simulink model "tractor_mu"  (R2022b)
settings: Solver=FixedStepDiscrete  StartTime=0.0  StopTime=20  FixedStep=0.001  RelTol=1e-3
model workspace (MAT data in the model file):
  P : object (value not decoded)
  w_2 : Simulink.Parameter (value not decoded)
undefined symbols (not defined in the file): A, a, B, b, C, D, DiscIntNeverNeededParam, Iz, K, k1, K1, k2, K2, L1, L2, m, magnitude, Phi, Sample_time, Steer_Ratio
libraries: simulink x26, slpidlib x13, Solver_SF x1, dsparch4 x1
(part 6 of 7)

== matlab function tractor_mu/加速度滑模观测/MATLAB Function1 ==
  data: a_xm input; a_xc output; a_ym input; v_xGPS input; v_yGPS input; gamma_c input; GPS_update_flag input; a_yc output; e_ax_est output; e_ay_est output; reset input
function [a_xc, a_yc, e_ax_est, e_ay_est] = accel_SMO_correction(a_xm, a_ym, v_xGPS, v_yGPS, gamma_c, GPS_update_flag, reset)
% 加速度滑模观测器校正
% 输入：
%   a_xm, a_ym      - INS测量的加速度 (m/s^2)
%   v_xGPS, v_yGPS  - GPS测量的速度 (m/s)
%   gamma_c         - 校正后的横摆角速度 (rad/s)
%   GPS_update_flag - GPS更新标志 (1=有新数据)
%   reset           - 复位信号
% 输出：
%   a_xc, a_yc      - 校正后的加速度
%   e_ax_est, e_ay_est - 估计的加速度偏差

% 采样时间
dt = 0.001;     % 仿真步长
DT = 0.05;      % GPS采样周期

% 滑模观测器增益（需根据实际调参）
persistent k1 k2 lambda1 lambda2
if isempty(k1)
    k1 = 5;       % 速度误差增益
    k2 = 5;
    lambda1 = 0.5; % 加速度偏差增益
    lambda2 = 0.5;
end

% 持久变量（状态记忆）
persistent v_xI v_yI e_ax e_ay initialized
persistent a_xm_sum a_ym_sum sum_count

if isempty(initialized) || reset
    v_xI = 0;      % INS积分速度 x
    v_yI = 0;      % INS积分速度 y
    e_ax = 0;      % 加速度偏差估计 x
    e_ay = 0;      % 加速度偏差估计 y
    a_xm_sum = 0;  % 加速度累加（用于GPS周期内求和）
    a_ym_sum = 0;
    sum_count = 0;
    initialized = true;
end

% 累加加速度（对应论文中的求和项）
a_xm_sum = a_xm_sum + a_xm;
a_ym_sum = a_ym_sum + a_ym;
sum_count = sum_count + 1;

% 速度积分（考虑横摆角速度耦合，对应式3-10）
% v_xI(k+1) = v_xI(k) + dt*a_xm + DT*(v_yI*gamma_c - e_ax - n_ax)
% 简化：每步用校正后的加速度积分
a_xc_temp = a_xm - e_ax;
a_yc_temp = a_ym - e_ay;

% 考虑横摆角速度耦合的速度更新
v_xI = v_xI + dt * (a_xc_temp + v_yI * gamma_c);
v_yI = v_yI + dt * (a_yc_temp - v_xI * gamma_c);

% GPS更新时刻：执行滑模校正
if GPS_update_flag == 1
    % 速度误差（观测残差）
    e_vx = v_xI - v_xGPS;
    e_vy = v_yI - v_yGPS;
    
    % 滑模切换函数
    s_x = sign(e_vx);
    s_y = sign(e_vy);
    
    % 也可用饱和函数避免抖振
    % epsilon = 0.1;
    % s_x = sat_func(e_vx, epsilon);
    % s_y = sat_func(e_vy, epsilon);
    
    % 速度校正（直接用GPS速度重置，或软校正）
    % 软校正方式：
    v_xI = v_xI - k1 * DT * s_x;
    v_yI = v_yI - k2 * DT * s_y;
    
    % 加速度偏差更新（滑模观测器核心）
    e_ax = e_ax + lambda1 * DT * s_x;
    e_ay = e_ay + lambda2 * DT * s_y;
    
    % 限幅防止发散
    e_ax = max(min(e_ax, 2), -2);
    e_ay = max(min(e_ay, 2), -2);
    
    % 清零累加器
    a_xm_sum = 0;
    a_ym_sum = 0;
    sum_count = 0;
end

% 输出校正后的加速度（式3-12）
a_xc = a_xm - e_ax;
a_yc = a_ym - e_ay;

% 输出偏差估计（用于调试）
e_ax_est = e_ax;
e_ay_est = e_ay;

end

% 饱和函数（可选，减少抖振）
function y = sat_func(x, epsilon)
    if abs(x) <= epsilon
        y = x / epsilon;
    else
        y = sign(x);
    end
end

== matlab function tractor_mu/质心侧偏角观测/MATLAB Function ==
  data: x_hat input; x_dot output; u input; z_meas input; z_hat output
function [x_dot, z_hat] = fcn(x_hat, u, z_meas)

    % === 车辆物理参数 ===
    mv = 18530;       % Vehicle total mass (kg)
    Izz = 67536;      % Second moment of mass (kg m^2)
    L1 = 2.043;        % CG to front axle (m)
    L2 = 1.362;        % CG to rear axle (m)
    Cf1 = 304828 * 2;     % Front cornering stiffness (N/rad) - 对应图中 C_F\delta^1
    Cf2 = 417040 * 2;     % Rear cornering stiffness (N/rad) - 对应图中 C_F\delta^2

    % === 观测器参数===
    Lambda = [100, 0;    % 增益矩阵 (3x2)
          0, 100;    
          0, 1000];   
    lambda_param = 1;
    Ts = 0.001;           % 离散采样时间 (Discrete Sample Time)

    % === 1. 解包状态变量和输入 ===
    % x_hat = [Vg_est; delta_est; r_est] 
    x1 = x_hat(1); % V_G
    x2 = x_hat(2); % delta (侧偏角)
    x3 = x_hat(3); % psi_dot (横摆角速度)

    % u = [beta; Fl1; Fl2]
    u1 = u(1); % beta
    u2 = u(2); % Fl1
    u3 = u(3); % Fl2
    
    % 防止分母为0
    if abs(x1) < 0.1
        x1 = 0.1; 
    end

    % === 2. 计算估计的输出 z_hat  ===
    % z = [Vg; psi_dot]
    h_NL = [x1; x3]; 
    z_hat = h_NL;

    % === 3. 计算观测误差 (z - z_hat) ===
    error = z_meas - z_hat;

    % === 4. 计算 Sign_eq 函数 ===
    sign_term = (2/pi) * atan(lambda_param * error);

    % === 5. 计算非线性函数 ===
    term1_1 = (1/mv) * (u2 * cos(x2 - u1) + u3 * cos(x2));
    term1_2 = (1/mv) * Cf2 * (-x2 + L2*x3/x1) * sin(x2);
    term1_3 = (1/mv) * Cf1 * (u1 - x2 - L1*x3/x1) * sin(x2 - u1);
    
    dx1_val = term1_1 + term1_2 + term1_3;

    term2_1 = 1/(mv*x1) * (u2 * sin(u1 - x2) - u3 * sin(x2)) ;
    term2_2 = 1/(mv*x1) * Cf1 * (u1 - x2 - L1*x3/x1) * cos(u1 - x2);
    term2_3 = 1/(mv*x1) * Cf2 * (-x2 + L2*x3/x1) * cos(x2) - x3;
    
    dx2_val = term2_1 + term2_2 + term2_3;

    term3_1 = (1/Izz) * ( L1 * u2 * sin(u1) - L2 * Cf2 * (-x2 + L2*x3/x1) ); 
    term3_2 = (1/Izz) * L1 * Cf1 * (u1 - x2 - L1*x3/x1) * cos(u1);
    
    dx3_val = term3_1 + term3_2;
    
    f_NL = [dx1_val; dx2_val; dx3_val];

    % === 6. 最终观测器状态导数 ===
    % x_hat_dot = f_NL(x_hat, u) + Lambda * sign_eq(z - z_hat)
    x_dot = f_NL + Lambda * sign_term;
end

== matlab function tractor_mu/软土扭矩分配/牵引功率目标计算 ==
  data: dt_s input; drawbar_power_w output; wheel_omegas_radps input; previous_applied_torques_n_m input; longitudinal_speed_mps input; implement_force_x_n input; wheel_power_w output; phi_raw output; filtered_phi output; filtered_normalized_phi output; lambda_est output; objective_valid output
function [drawbar_power_w, wheel_power_w, phi_raw, filtered_phi, filtered_normalized_phi, lambda_est, objective_valid] = MF_TractionEfficiencyObjective(dt_s, wheel_omegas_radps, previous_applied_torques_n_m, longitudinal_speed_mps, implement_force_x_n)

% 牵引效率目标函数计算模块
%
% 本模块计算牵引效率相关的在线优化目标：
% eta = P_drawbar / P_wheel
%
% 并构造 Dinkelbach 差值型目标：
% phi = P_drawbar - lambda * P_wheel

persistent has_filtered_power filtered_drawbar_power_state filtered_wheel_power_state
persistent has_filtered_phi filtered_phi_state filtered_normalized_phi_state
persistent lambda_state

if isempty(has_filtered_power)

    has_filtered_power = 0.0;
    filtered_drawbar_power_state = 0.0;
    filtered_wheel_power_state = 0.0;

    has_filtered_phi = 0.0;
    filtered_phi_state = 0.0;
    filtered_normalized_phi_state = 0.0;

    lambda_state = 0.0;
end

%% 输入整理

dt = max(double(dt_s), 0.0);
omegas = row4_local(wheel_omegas_radps);
applied_torques = row4_local(previous_applied_torques_n_m);

vx = double(longitudinal_speed_mps);
implement_force = double(implement_force_x_n);

%% 轮端输入功率计算

% 轮端输入功率 P_wheel = sum(T_i * omega_i)。
% 只保留非负驱动功率，避免制动功率或异常信号影响牵引效率评价。
wheel_drive_powers = zeros(1, 4);

for index = 1:4
    wheel_drive_powers(index) = max(0.0, applied_torques(index) * abs(omegas(index)));
end

wheel_power_w = sum(wheel_drive_powers);

%% 有效牵引功率计算

% 农具阻力方向通常与车辆行驶方向相反。
% 前进时，如果 implement_force 为负，则 -implement_force 为有效牵引阻力。
% 倒车时符号相反。
if vx > 0.08
    drawbar_force = max(0.0, -implement_force);
elseif vx < -0.08
    drawbar_force = max(0.0, implement_force);
else
    drawbar_force = 0.0;
end

drawbar_power_w = drawbar_force * abs(vx);

%% 目标函数有效性判断

% 轮端输入功率过低或车速过低时，牵引效率计算不可靠。
objective_valid = wheel_power_w >= 100.0 && abs(vx) > 0.08;

%% 功率滤波

alpha_objective = first_order_alpha_local(dt, 0.7);

if has_filtered_power <= 0.5 || ~objective_valid

    filtered_drawbar_power_state = drawbar_power_w;
    filtered_wheel_power_state = wheel_power_w;
    has_filtered_power = 1.0;

else

    filtered_drawbar_power_state = filtered_drawbar_power_state + ...
        alpha_objective * (drawbar_power_w - filtered_drawbar_power_state);

    filtered_wheel_power_state = filtered_wheel_power_state + ...
        alpha_objective * (wheel_power_w - filtered_wheel_power_state);

    has_filtered_power = 1.0;
end

%% lambda 牵引效率参数更新

if objective_valid

    eta_instant = drawbar_power_w / max(wheel_power_w, 1.0e-9);

    alpha_lambda = first_order_alpha_local(dt, 1.0);

    lambda_state = lambda_state + alpha_lambda * (eta_instant - lambda_state);
end

lambda_est = lambda_state;

%% Dinkelbach 差值型性能指标

phi_raw = drawbar_power_w - lambda_est * wheel_power_w;

% 归一化性能指标，用于降低功率量级变化对极值寻优的影响。
normalized_phi = phi_raw / max(abs(wheel_power_w), 1000.0);

%% 性能指标滤波

if has_filtered_phi <= 0.5 || ~objective_valid

    filtered_phi_state = phi_raw;
    filtered_normalized_phi_state = normalized_phi;
    has_filtered_phi = 1.0;

else

    filtered_phi_state = filtered_phi_state + ...
        alpha_objective * (phi_raw - filtered_phi_state);

    filtered_normalized_phi_state = filtered_normalized_phi_state + ...
        alpha_objective * (normalized_phi - filtered_normalized_phi_state);

    has_filtered_phi = 1.0;
end

filtered_phi = filtered_phi_state;
filtered_normalized_phi = filtered_normalized_phi_state;

end


function output = row4_local(values)

% 将输入信号整理为 1×4 行向量。

input_values = double(values);
output = zeros(1, 4);

for index = 1:4
    output(index) = input_values(index);
end

end


function alpha = first_order_alpha_local(dt, time_constant_s)

% 一阶低通滤波系数：
% y(k) = y(k-1) + alpha * [u(k) - y(k-1)]

if dt <= 0.0 || time_constant_s <= 0.0
    alpha = 1.0;
else
    alpha = dt / (time_constant_s + dt);
end

end

== matlab function tractor_mu/软土扭矩分配/四轮目标滑移率计算 ==
  data: current_time_s input; adaptive_targets output; dt_s input; filtered_normalized_phi input; objective_valid input; kappa_valid input; target_base_out output; gradient_estimates output
function [adaptive_targets, target_base_out, gradient_estimates] = MF_AdaptiveSlipTarget4W(current_time_s, dt_s, filtered_normalized_phi, objective_valid, kappa_valid)

% 四轮自适应目标滑移率生成模块
%
% 采用多变量极值寻优思想，对四个车轮的目标滑移率进行独立更新。
%
% 四轮顺序：
% 1：左前轮
% 2：右前轮
% 3：左后轮
% 4：右后轮

persistent target_base_state gradient_state

if isempty(target_base_state)

    % 初始目标滑移率仍保持原前后轴标定值。
    target_base_state = [0.078, 0.078, 0.128, 0.128];

    % 四轮梯度估计初值。
    gradient_state = zeros(1, 4);
end

%% 输入整理

time_s = double(current_time_s);
dt = max(double(dt_s), 0.0);
normalized_phi = double(filtered_normalized_phi);
valid_vec = row4_local(kappa_valid);

%% 极值寻优参数

% 四轮扰动频率，单位 Hz。
frequencies = [0.7, 0.9, 1.1, 1.3];

% 目标滑移率扰动幅值。
perturb_amp = 0.002;

% 目标滑移率基值自适应增益。
adapt_gain = 0.0006;

% 目标滑移率允许范围。
target_min = 0.03;
target_max = 0.25;

% 梯度低通滤波系数。
alpha_gradient = first_order_alpha_local(dt, 0.8);

%% 是否允许更新目标基值

update_enabled = double(objective_valid) > 0.5 && all(valid_vec > 0.5);

%% 生成四轮扰动信号

sine_signals = zeros(1, 4);

for index = 1:4
    sine_signals(index) = sin(2.0 * pi * frequencies(index) * time_s);
end

%% 梯度估计与目标基值更新

if update_enabled

    for index = 1:4

        % 极值寻优解调。
        % 性能指标与扰动信号相乘，用于估计该轮目标滑移率变化对牵引效率目标的边际影响。
        gradient_raw = 2.0 * normalized_phi * sine_signals(index) / perturb_amp;

        % 梯度估计低通滤波。
        gradient_state(index) = gradient_state(index) + ...
            alpha_gradient * (gradient_raw - gradient_state(index));

        % 限制每个采样周期目标滑移率基值的最大变化量。
        max_delta = 0.003 * dt;

        target_delta = clamp_local(adapt_gain * gradient_state(index) * dt, -max_delta, max_delta);

        % 更新目标滑移率基值。
        target_base_state(index) = clamp_local(target_base_state(index) + target_delta, target_min, target_max);
    end
end

%% 输出四轮目标滑移率

adaptive_targets = zeros(1, 4);

for index = 1:4

    % 最终目标 = 基值 + 小幅正弦扰动。
    adaptive_targets(index) = clamp_local( ...
        target_base_state(index) + perturb_amp * sine_signals(index), ...
        target_min, target_max);
end

% 调试输出，可在 Simulink 中不连接。
target_base_out = target_base_state;
gradient_estimates = gradient_state;

end


function output = row4_local(values)

% 将输入信号整理为 1×4 行向量。

input_values = double(values);
output = zeros(1, 4);

for index = 1:4
    output(index) = input_values(index);
end

end


function alpha = first_order_alpha_local(dt, time_constant_s)

% 一阶低通滤波系数。

if dt <= 0.0 || time_constant_s <= 0.0
    alpha = 1.0;
else
    alpha = dt / (time_constant_s + dt);
end

end


function value = clamp_local(value_in, lower, upper)

% 数值限幅函数。

value = min(max(double(value_in), double(lower)), double(upper));

end

== matlab function tractor_mu/牵引效率计算/计算平均边际贡献 ==
  data: v_all input; phi output
function phi = shapley_calc(v_all)

% 输入:
% v_all: 16x1
%
% 子集顺序:
%
% 1  -> []
% 2  -> [1]
% 3  -> [2]
% 4  -> [3]
% 5  -> [4]
% 6  -> [1 2]
% 7  -> [1 3]
% 8  -> [1 4]
% 9  -> [2 3]
% 10 -> [2 4]
% 11 -> [3 4]
% 12 -> [1 2 3]
% 13 -> [1 2 4]
% 14 -> [1 3 4]
% 15 -> [2 3 4]
% 16 -> [1 2 3 4]
%
% 输出:
% phi = [FL; FR; RL; RR]

%% 平移法消除负值

v_min = min(v_all);

if v_min < 0
    v_all = v_all - v_min;
end

%% 参数

n = 4;

fact = factorial(0:n);

phi = zeros(4,1);

%% 联盟定义

coalitions = [...
    0 0 0 0;  % 1
    1 0 0 0;  % 2
    0 1 0 0;  % 3
    0 0 1 0;  % 4
    0 0 0 1;  % 5
    1 1 0 0;  % 6
    1 0 1 0;  % 7
    1 0 0 1;  % 8
    0 1 1 0;  % 9
    0 1 0 1;  % 10
    0 0 1 1;  % 11
    1 1 1 0;  % 12
    1 1 0 1;  % 13
    1 0 1 1;  % 14
    0 1 1 1;  % 15
    1 1 1 1]; % 16

%% Shapley计算

for i = 1:n

    for idx = 1:16

        S = coalitions(idx,:);

        % 若联盟中已有玩家i
        if S(i) == 1
            continue;
        end

        % 联盟大小
        k = sum(S);

        % 权重
        w = fact(k+1) * fact(n-k) / fact(n+1);

        % v(S)
        v_S = v_all(idx);

        % 构造 S∪{i}
        S_with_i = S;
        S_with_i(i) = 1;

        %% 查找 S∪{i} 对应索引

        idx_Si = 1;

        for j = 1:16

            if isequal(coalitions(j,:), S_with_i)

                idx_Si = j;
                break;

            end

        end

        % v(S∪{i})
        v_Si = v_all(idx_Si);

        % Shapley累加
        phi(i) = phi(i) + w * (v_Si - v_S);

    end

end

phi_min = min(phi);

if phi_min < 0
    phi = phi - phi_min;
end

end

== matlab function tractor_mu/协同博弈扭矩分配/MATLAB Function ==
  data: v input; alpha output
function alpha = fcn(v)

if v < 0.5
    alpha = 0;
elseif v < 5
    alpha = (v - 0.5)/(5 - 0.5);
else
    alpha = 1;
end

== matlab function tractor_mu/牵引效率计算/MATLAB Function3 ==
  data: Fx input; V_all output; Vx input; T input; uF input; mu input; Fz input; slip input; Mz_ref input; Traction_all output; lamdaN_all output; lamda_all output; Mz_all output
function [V_all,Traction_all,lamdaN_all,lamda_all,Mz_all] = shapley_value_all(...
Fx,...
Vx,...
T,...
uF,...
mu,...
Fz,...
slip,...
Mz_ref)

%% 参数

kf = 3;   % 前轮牵引权重
kr = 6;   % 后轮牵引权重

w1 = 100000;  % 滑转率损失权重
w2 = 5000;    % 附着利用率均衡权重
w3 = 0.0001;  % 横摆稳定损失权重

% 半轮距
bf = 2.39/2;
br = 2.33/2;

%% 初始化

V_all = zeros(16,1);
Traction_all = zeros(16,1);
lamdaN_all = zeros(16,1);
lamda_all = zeros(16,1);
Mz_all = zeros(16,1);

%% 16个联盟

coalitions = [...
    0 0 0 0;  % 空集-1
    1 0 0 0;  % 2
    0 1 0 0;  % 3
    0 0 1 0;  % 4
    0 0 0 1;  % 5
    1 1 0 0;  % 6
    1 0 1 0;  % 7
    1 0 0 1;  % 8
    0 1 1 0;  % 9
    0 1 0 1;  % 10
    0 0 1 1;  % 11
    1 1 1 0;  % 12
    1 1 0 1;  % 13
    1 0 1 1;  % 14
    0 1 1 1;  % 15
    1 1 1 1];  % 16

%% 遍历所有联盟

for k = 1:16

    coalition = coalitions(k,:)';

    %% 联盟数据

    Fx_s    = Fx    .* coalition;
    T_s     = T     .* coalition;
    uF_s    = uF   .* coalition;
    mu_s    = mu    .* coalition;
    Fz_s    = Fz    .* coalition;
    slip_s  = slip   .* coalition;

    %% 1 牵引能力项

    F_front = uF_s(1) + uF_s(2);
    F_rear  = uF_s(3) + uF_s(4);

    traction_term = ...
        kf * F_front + ...
        kr * F_rear;

    %% 2 滑转率损失

    
    % 只保留联盟中的驱动轮滑转率
    slip_active = abs(slip_s);

    % 防止空集导致 max([]) 问题
if sum(coalition) == 0

    lamdaN = 0;

else

    % 最大滑转率
    slip_max = max(slip_active);

    % 四次方强化惩罚
    lamdaN = slip_max^4;

end


    %% 3 附着利用率

    lambda_term = 0;

    for i = 1:4

        if coalition(i) == 1

            denom = uF_s(i);

            if abs(denom) > 1e-6

                lambda_i = Fx_s(i) / denom;

                % 平方强化
                lambda_term = ...
                    lambda_term + lambda_i^2;

            end

        end

    end

    %% 4 横摆力矩

    Mz = ...
        (-Fx_s(1) + Fx_s(2)) * bf + ...
        (-Fx_s(3) + Fx_s(4)) * br;

    %Mz = 

    %% 5 价值函数

    V_all(k) = ...
        traction_term ...
        - w1 * lamdaN ...
        + w2 * lambda_term ...
        - w3 * (Mz - Mz_ref)^2;

    Traction_all(k) = traction_term;
    lamdaN_all(k) = -w1 * lamdaN;
    lamda_all(k) = w2 * lambda_term;
    Mz_all(k) = - w3 * (Mz - Mz_ref)^2;

end

end

== matlab function tractor_mu/软土分配策略/MATLAB Function ==
  data: wheel_speeds_rpm input; selected_torques_n_m output; front_steer_angles_deg input; longitudinal_speed_mps input; applied_torques_n_m input; drive_torque_enabled input; baseline_torques_n_m input; wheel_torque_limits_n_m input; control_kappa output; filtered_kappa output; kappa_valid output; adaptive_targets output; cbf_torque_upper_bounds output; cbf_active output; nominal_torques_n_m output; soft_diag output
function [selected_torques_n_m, control_kappa, filtered_kappa, kappa_valid, adaptive_targets, cbf_torque_upper_bounds, cbf_active, nominal_torques_n_m, soft_diag] = shiche_soft_soil_adaptive_allocation(wheel_speeds_rpm, front_steer_angles_deg, longitudinal_speed_mps, applied_torques_n_m, drive_torque_enabled, baseline_torques_n_m, wheel_torque_limits_n_m)
%SHICHE_SOFT_SOIL_ADAPTIVE_ALLOCATION Real-vehicle soft-soil clamp allocator.
%
% MATLAB Function block version for VCU code generation. All numeric states,
% constants, intermediate arrays, and outputs are single precision.
%
% Wheel vector order is fixed as a 4x1 column:
%   [L1, R1, L2, R2] = [left-front, right-front, left-rear, right-rear]
%
% This block assumes an upstream load-based/basic four-wheel torque allocator
% already exists. baseline_torques_n_m is used as the reproducible anchor
% allocation. This real-vehicle version intentionally avoids QP, matrix solves,
% and active-set enumeration: it applies slip-tracking torque correction and
% then clamps each wheel by the CBF safety upper bound.
%
% Inputs:
%   wheel_speeds_rpm        single, 4x1 wheel speeds in rpm, [L1 R1 L2 R2].
%   front_steer_angles_deg  single, [Steer_L1 Steer_R1] in deg, or one scalar.
%   longitudinal_speed_mps  single, vehicle longitudinal speed in m/s.
%   applied_torques_n_m     single, 4x1 actual or one-step delayed applied wheel
%                           torques in N*m, [L1 R1 L2 R2].
%   drive_torque_enabled    single flag, >0.5 enables adaptive update and CBF.
%   baseline_torques_n_m    single, 4x1 upstream basic allocation in N*m.
%   wheel_torque_limits_n_m single, 4x1 nonnegative wheel torque limits in N*m.
%
% Outputs are single. kappa_valid and cbf_active are 0/1 single flags. soft_diag
% has 26 entries:
%   1:6   front target, rear target, simplified allocator status, total torque
%         reduction by CBF clamp, baseline total torque, selected total torque
%   7:10  filtered slip derivatives
%   11:14 slip input gains
%   15:18 slip disturbance estimates
%   19:22 disturbance margins
%   23:26 wheel surface speeds

persistent has_filtered filtered_state filtered_dot_state disturbance_state

if isempty(has_filtered)
    has_filtered = zeros(4, 1, 'single');
    filtered_state = zeros(4, 1, 'single');
    filtered_dot_state = zeros(4, 1, 'single');
    disturbance_state = zeros(4, 1, 'single');
end

dt = single(0.02);
wheel_speeds = column4_local(wheel_speeds_rpm);
front_steers = front_steer_pair_local(front_steer_angles_deg);
control_vx = single(longitudinal_speed_mps);
applied_torques = column4_local(applied_torques_n_m);
base_torques = column4_local(baseline_torques_n_m);
wheel_limits = column4_local(wheel_torque_limits_n_m);
drive_enabled = single(drive_torque_enabled) > single(0.5);

for index = 1:4
    wheel_limits(index) = max(single(0.0), wheel_limits(index));
    base_torques(index) = clamp_local(base_torques(index), single(0.0), wheel_limits(index));
end

[control_kappa, filtered_kappa, kappa_valid, dot_kappa, rolling_speeds, wheel_omegas, surface_speeds, has_filtered, filtered_state, filtered_dot_state] = ...
    update_slip_local(wheel_speeds, front_steers, control_vx, dt, has_filtered, filtered_state, filtered_dot_state);

front_target_base = single(0.078);
rear_target_base = single(0.128);
adaptive_targets = zeros(4, 1, 'single');
adaptive_targets(1) = front_target_base;
adaptive_targets(2) = front_target_base;
adaptive_targets(3) = rear_target_base;
adaptive_targets(4) = rear_target_base;

input_gains = input_gains_local(kappa_valid, rolling_speeds, wheel_omegas);
[disturbance_state, disturbance_margins] = update_disturbance_local(kappa_valid, dot_kappa, input_gains, applied_torques, dt, disturbance_state);

front_error = axle_slip_error_local(filtered_kappa, kappa_valid, adaptive_targets(1), 1);
rear_error = axle_slip_error_local(filtered_kappa, kappa_valid, adaptive_targets(3), 2);

nominal_torques_n_m = zeros(4, 1, 'single');
cbf_torque_upper_bounds = zeros(4, 1, 'single');
cbf_active = zeros(4, 1, 'single');
for index = 1:4
    gain = input_gains(index);
    if drive_enabled && kappa_valid(index) > single(0.5) && isfinite(gain)
        if index <= 2
            axle_error = front_error;
        else
            axle_error = rear_error;
        end
        torque_delta = clamp_local(-single(20500.0) * axle_error, -single(2600.0), single(2600.0));
        nominal = base_torques(index) + torque_delta;
    else
        nominal = base_torques(index);
    end
    nominal_torques_n_m(index) = clamp_local(nominal, single(0.0), wheel_limits(index));

    if drive_enabled && kappa_valid(index) > single(0.5) && isfinite(gain)
        upper = (single(15.0) * (single(0.25) - filtered_kappa(index)) - disturbance_state(index) - disturbance_margins(index)) / gain;
        if ~isfinite(upper)
            upper = wheel_limits(index);
        end
        upper = clamp_local(upper, single(0.0), wheel_limits(index));
    else
        upper = wheel_limits(index);
    end
    cbf_torque_upper_bounds(index) = upper;
    if upper < base_torques(index) - single(1.0e-6)
        cbf_active(index) = single(1.0);
    end
end

selected_torques_n_m = zeros(4, 1, 'single');
for index = 1:4
    selected_torques_n_m(index) = clamp_local(nominal_torques_n_m(index), single(0.0), cbf_torque_upper_bounds(index));
end

allocator_status = single(1.0);
total_torque_reduction = sum(nominal_torques_n_m - selected_torques_n_m);
baseline_total_torque = sum(base_torques);
selected_total_torque = sum(selected_torques_n_m);

soft_diag = zeros(26, 1, 'single');
soft_diag(1) = front_target_base;
soft_diag(2) = rear_target_base;
soft_diag(3) = allocator_status;
soft_diag(4) = total_torque_reduction;
soft_diag(5) = baseline_total_torque;
soft_diag(6) = selected_total_torque;
for index = 1:4
    soft_diag(6 + index) = dot_kappa(index);
    soft_diag(10 + index) = input_gains(index);
    soft_diag(14 + index) = disturbance_state(index);
    soft_diag(18 + index) = disturbance_margins(index);
    soft_diag(22 + index) = surface_speeds(index);
end
end

function [raw_kappa, filtered_kappa, valid, dot_kappa, rolling_speeds, omegas, surface_speeds, has_filtered_out, filtered_state_out, filtered_dot_out] = update_slip_local(wheel_speeds, front_steers, vx_mps, dt, has_filtered_in, filtered_state_in, filtered_dot_in)
rpm_to_rad = single(2.0) * single(pi) / single(60.0);
radii = zeros(4, 1, 'single');
radii(1) = single(0.834);
radii(2) = single(0.834);
radii(3) = single(0.94);
radii(4) = single(0.94);
speed_abs = abs(single(vx_mps));
steer_l = front_steers(1) * single(pi) / single(180.0);
steer_r = front_steers(2) * single(pi) / single(180.0);
rolling_speeds = zeros(4, 1, 'single');
rolling_speeds(1) = abs(speed_abs * cos(steer_l));
rolling_speeds(2) = abs(speed_abs * cos(steer_r));
rolling_speeds(3) = speed_abs;
rolling_speeds(4) = speed_abs;
omegas = abs(single(wheel_speeds)) * rpm_to_rad;
surface_speeds = radii .* omegas;

raw_kappa = zeros(4, 1, 'single');
filtered_kappa = zeros(4, 1, 'single');
dot_kappa = zeros(4, 1, 'single');
valid = zeros(4, 1, 'single');
has_filtered_out = has_filtered_in;
filtered_state_out = filtered_state_in;
filtered_dot_out = filtered_dot_in;
for index = 1:4
    raw_kappa(index) = single(NaN);
    filtered_kappa(index) = single(NaN);
end

alpha_kappa = first_order_alpha_local(dt, single(0.04));
alpha_dot = first_order_alpha_local(dt, single(0.08));
for index = 1:4
    is_valid = speed_abs >= single(0.08) && surface_speeds(index) >= single(0.20) && isfinite(rolling_speeds(index)) && isfinite(surface_speeds(index));
    if is_valid
        valid(index) = single(1.0);
        raw_value = single(1.0) - rolling_speeds(index) / surface_speeds(index);
        raw_kappa(index) = clamp_local(raw_value, -single(1.0), single(1.0));
        if has_filtered_in(index) <= single(0.5) || ~isfinite(filtered_state_in(index))
            filtered_value = raw_kappa(index);
            raw_dot = single(0.0);
        else
            previous = filtered_state_in(index);
            filtered_value = previous + alpha_kappa * (raw_kappa(index) - previous);
            raw_dot = (filtered_value - previous) / dt;
        end
        filtered_dot_out(index) = filtered_dot_in(index) + alpha_dot * (raw_dot - filtered_dot_in(index));
        filtered_state_out(index) = filtered_value;
        has_filtered_out(index) = single(1.0);
        filtered_kappa(index) = filtered_value;
        dot_kappa(index) = filtered_dot_out(index);
    else
        if has_filtered_in(index) > single(0.5)
            raw_kappa(index) = filtered_state_in(index);
            filtered_kappa(index) = filtered_state_in(index);
        end
        filtered_dot_out(index) = single(0.0);
        dot_kappa(index) = single(0.0);
    end
end
end

function front_steers = front_steer_pair_local(front_steer_angles_deg)
% Accept [Steer_L1, Steer_R1] or one equivalent front-axle steer angle.
steer_input = single(front_steer_angles_deg);
front_steers = zeros(2, 1, 'single');
if numel(steer_input) >= 2
    front_steers(1) = steer_input(1);
    front_steers(2) = steer_input(2);
else
    front_steers(1) = steer_input(1);
    front_steers(2) = steer_input(1);
end
end

function gains = input_gains_local(valid, rolling_speeds, omegas)
radii = zeros(4, 1, 'single');
radii(1) = single(0.834);
radii(2) = single(0.834);
radii(3) = single(0.94);
radii(4) = single(0.94);
inertias = zeros(4, 1, 'single');
inertias(1) = single(450.0);
inertias(2) = single(450.0);
inertias(3) = single(650.0);
inertias(4) = single(650.0);
gains = zeros(4, 1, 'single');
for index = 1:4
    gains(index) = single(NaN);
end
for index = 1:4
    if valid(index) > single(0.5) && omegas(index) > single(0.0)
        gain = rolling_speeds(index) / (inertias(index) * radii(index) * omegas(index) * omegas(index));
        if gain >= single(1.0e-8)
            gains(index) = gain;
        end
    end
end
end

function [disturbance_out, margins] = update_disturbance_local(valid, dot_kappa, input_gains, applied_torques, dt, disturbance_in)
disturbance_out = disturbance_in;
margins = zeros(4, 1, 'single');
alpha_disturbance = first_order_alpha_local(dt, single(0.15));
for index = 1:4
    gain = input_gains(index);
    if valid(index) > single(0.5) && isfinite(gain)
        raw_estimate = dot_kappa(index) - gain * applied_torques(index);
        disturbance_out(index) = disturbance_in(index) + alpha_disturbance * (raw_estimate - disturbance_in(index));
        residual = raw_estimate - disturbance_out(index);
    else
        residual = single(0.0);
    end
    margins(index) = clamp_local(single(0.05) + single(0.05) * abs(residual), single(0.05), single(5.0));
end
end

function error = axle_slip_error_local(filtered_kappa, valid, target, axle_id)
total = single(0.0);
count = single(0.0);
if axle_id == 1
    start_index = 1;
    end_index = 2;
else
    start_index = 3;
    end_index = 4;
end
for index = start_index:end_index
    if valid(index) > single(0.5) && isfinite(filtered_kappa(index))
        total = total + filtered_kappa(index);
        count = count + single(1.0);
    end
end
if count > single(0.0)
    error = total / count - target;
else
    error = single(0.0);
end
end

function alpha = first_order_alpha_local(dt, time_constant_s)
if dt <= single(0.0) || time_constant_s <= single(0.0)
    alpha = single(1.0);
else
    alpha = dt / (time_constant_s + dt);
end
end

function value = clamp_local(value_in, lower, upper)
value = min(max(single(value_in), single(lower)), single(upper));
end

function output = column4_local(values)
input_values = single(values);
output = zeros(4, 1, 'single');
for index = 1:4
    output(index) = input_values(index);
end
end

== stateflow chart tractor_mu/总驱动力矩制定/负载工况_极限防抖 ==
  state Normal
    entry:
    T_hold = 0;
    during:
    T0_out = T0;
  state Limit_detect
    during:
    T0_out = T0;
  state Limit_hold
    entry:
    T_hold = T0;
    during:
    T_hold = T_hold + 0.02*(T0 - T_hold);
    T_hold = min(max(T_hold,2000),60000);
    T0_out = T_hold;
  (default) -> Normal
  Limit_detect -> Normal [order 1] : [(throttle < 0.7) || (load_rate < 0.9) || (abs(ax) > 0.1)]
  Normal -> Limit_detect : [(throttle > 0.8) && (load_rate > 0.9) && (abs(ax) < 0.1) ]
  Limit_hold -> Normal : [ (load_rate < 0.85) && (abs(ax) > 0.12)]
  Limit_detect -> Limit_hold [order 2] : [after(0.5,sec)]
  data: throttle input; ax input; Tmax input; load_rate input; T0 input; T0_out output; T_hold local; timer_start local

== matlab function tractor_mu/PID_Controller//直线循迹/MATLAB Function ==
  data: u input; y output
function y = lowpass_filter(u)
persistent prev_x prev_y;
if isempty(prev_x), prev_x = 0; end
if isempty(prev_y), prev_y = 0; end

% 差分方程: y(n) = 0.2452*u(n) + 0.2452*u(n-1) + 0.5095*y(n-1)
y = 0.2452*u + 0.2452*prev_x + 0.5095*prev_y;

% 更新状态
prev_x = double(u);
prev_y = double(y);
end

== matlab function tractor_mu/PID_Controller//直线循迹/MATLAB Function2 ==
  data: st input; flag_ctrl output; flag_cnt output; yaw input; throttle input; yaw_ref output
function [flag_ctrl, flag_cnt, yaw_ref] = StraightModeDetector(st, yaw, throttle)

%% 实车调试版本
% 所有 persistent 变量必须为 single 以满足实车要求 
persistent ctrl_cnt yaw_sum yaw_time yaw_ref_int yaw_f
if isempty(ctrl_cnt)
    ctrl_cnt    = single(0);
    yaw_sum     = single(0);
    yaw_time    = single(0);
    yaw_ref_int = single(0);
    yaw_f       = single(0);
end

%% === 参数 ===
st_lim_enter = single(1);     % 进入判定阈值 (deg)
st_lim_exit  = single(1.2);     % 退出判定（滞回）
thr_min      = single(1);       % 油门下限 (%)
thr_max      = single(50);      % 油门上限 (%)


T_ctrl   = single(3.0);         % 需要检测的直行时间 (s)
Ts       = single(0.02);        % sample time
num_ctrl = single(T_ctrl / Ts); % 循环次数

alpha = single(0.15);           % LPF 低通滤波器系数
flag_cnt = single(0);           % 累加计算目标航向使能

%% === Step 1: LPF 过滤 yaw ===
yaw_f = yaw_f + alpha * (yaw - yaw_f);

%% === Step 2: 判断是否满足直行条件 ===
cond_enter = (abs(st) < st_lim_enter) && (throttle > thr_min) && (throttle < thr_max);
cond_exit  = (abs(st) > st_lim_exit)  || (throttle <= thr_min) || (throttle >= thr_max);

%% === Step 3: 计数器逻辑 ===
if cond_enter
    ctrl_cnt = ctrl_cnt + 1;
else
    ctrl_cnt = single(0);
end

%% === Step 4: yaw 采样（累加）===
if cond_enter && (ctrl_cnt <= num_ctrl)
    yaw_sum  = yaw_sum  + yaw_f;
    yaw_time = yaw_time + 1;
    flag_cnt = single(1);
end

%% === Step 5: 进入直线控制模式的瞬间冻结 yaw_ref ===
% if ctrl_cnt == num_ctrl
%     yaw_ref_int = yaw_sum / yaw_time;
% end
if (ctrl_cnt >= num_ctrl) && (yaw_time > 0) && (yaw_ref_int == 0)
    yaw_ref_int = yaw_sum / yaw_time;
end

%% === Step 6: 若退出模式，则清空状态 ===
if cond_exit
    ctrl_cnt    = single(0);
    yaw_sum     = single(0);
    yaw_time    = single(0);
    yaw_ref_int = single(0);
end

%% === Step 7: 输出 ===
flag_ctrl = single(ctrl_cnt >= num_ctrl);
yaw_ref   = yaw_ref_int;

end

== matlab function tractor_mu/PID_Controller//直线循迹/指数加权移动平均 ==
  data: uk input; y output; is_biased input

function y = ExpMovAvg(uk, is_biased)
% 指数加权移动平均滤波器
% 输入:
%   uk      : 当前输入值
%   is_biased: 是否应用偏差修正 (1=是, 0=否)
% 输出:
%   y       : 指数加权移动平均值

% 持久变量保持状态 (在时间步之间保留值)
persistent shadow count first_time decay

% 初始化参数和状态
if isempty(first_time)
    % 初始化标志
    first_time = true;
    
    % 初始化状态值
    shadow = double(0);
    count = 0;
    
    % 设置衰减因子 (0.9是常用值，可根据需要修改)
    decay = 0.9;
end

% 主处理逻辑
if first_time
    % 第一次调用 - 初始化状态
    shadow = double(uk);
    count = 1;
    first_time = false;
    y = uk;  % 第一次返回当前值
else
    % 更新计数器
    count = count + 1;
    
    % 计算指数加权平均值
     a = decay * shadow + (1 - decay) * uk;
    shadow = double(a);
    
    if is_biased
        % 应用偏差修正 (1 - decay^count)
        bias_correction = 1 - decay^count;
         b = shadow / bias_correction;
        y = single(b);
    else
        % 返回原始加权平均值
        y = single(shadow);
    end
end
end

== matlab function tractor_mu/PID_Controller//直线循迹/模式判断 ==
  data: v input; st input; avg input; mode output
function mode  = stateflow(v,st,avg)

mode = 7; %常规模式

% 沥青路面判断
    if avg <= 2
        if v > 20
            if st>=8
                mode = 1; % 高速转向
            elseif st<=3
                mode = 2; % 高速直行
            end
        elseif v < 10
            if st>=5
                mode = 3; % 低速转向
            elseif st<5
                mode = 4; % 低速直行
            end
        end
    % 土地路面判断
    elseif avg >= 3
        if v >= 10
            mode = 5; % 土地快速
        elseif v < 10
            mode = 6; % 土地低速
        end
    end
end

== matlab function tractor_mu/软土扭矩分配/滑移跟踪与扭矩生成 ==
  data: kappa input; nominal_torques_n_m output; kappa_valid input; input_gains input; adaptive_targets input; base_torques_n_m input; wheel_limits_n_m input; slip_errors output
function [nominal_torques_n_m, slip_errors] = MF_SlipTrackingNominalTorque(kappa, kappa_valid, input_gains, adaptive_targets, base_torques_n_m, wheel_limits_n_m)

% 滑移跟踪与名义扭矩生成模块
%
% 根据四轮实际滑移率与四轮目标滑移率之间的误差，生成名义轮端扭矩。
%
% 名义扭矩不是最终输出扭矩，后续还需要经过 CBF-QP 模块进行安全约束和协调分配。

%% 输入整理

kappa_vec = row4_local(kappa);
valid_vec = row4_local(kappa_valid);
gain_vec = row4_local(input_gains);
target_vec = row4_local(adaptive_targets);
base_vec = row4_local(base_torques_n_m);
limit_vec = row4_local(wheel_limits_n_m);

%% 控制参数

% 滑移率误差到扭矩修正的比例增益。
slip_tracking_gain = 20500.0;

% 单轮扭矩修正量限幅。
torque_delta_limit = 2600.0;

%% 四轮名义扭矩计算

nominal_torques_n_m = zeros(1, 4);
slip_errors = zeros(1, 4);

for index = 1:4

    wheel_limit = max(0.0, limit_vec(index));
    base_torque = clamp_local(base_vec(index), 0.0, wheel_limit);

    if valid_vec(index) > 0.5 && isfinite(kappa_vec(index)) && isfinite(target_vec(index)) && isfinite(gain_vec(index))

        % 四轮独立滑移率跟踪误差。
        slip_errors(index) = kappa_vec(index) - target_vec(index);

        % 滑移率反馈扭矩修正。
        % 若实际滑移率大于目标，误差为正，扭矩修正为负，降低驱动扭矩；
        % 若实际滑移率小于目标，误差为负，扭矩修正为正，提高驱动扭矩。
        torque_delta = -slip_tracking_gain * slip_errors(index);

        % 扭矩修正限幅。
        torque_delta = clamp_local(torque_delta, -torque_delta_limit, torque_delta_limit);

        nominal = base_torque + torque_delta;

    else

        % 滑移率或输入增益无效时，不做滑移反馈修正，保持基线扭矩。
        slip_errors(index) = 0.0;
        nominal = base_torque;
    end

    % 名义扭矩满足物理轮端限幅。
    nominal_torques_n_m(index) = clamp_local(nominal, 0.0, wheel_limit);
end

end


function output = row4_local(values)

% 将输入信号整理为 1×4 行向量。

input_values = double(values);
output = zeros(1, 4);

for index = 1:4
    output(index) = input_values(index);
end

end


function value = clamp_local(value_in, lower, upper)

% 数值限幅函数。

value = min(max(double(value_in), double(lower)), double(upper));

end

== matlab function tractor_mu/软土扭矩分配/CBF-QP扭矩分配 ==
  data: dt_s input; selected_torques_n_m output; kappa input; dot_kappa input; kappa_valid input; input_gains input; previous_applied_torques_n_m input; nominal_torques_n_m input; base_torques_n_m input; wheel_limits_n_m input; front_steers_rad input; total_torque_n_m input; control_mz_n_m input; cbf_torque_upper_bounds output; cbf_active output; qp_status output; qp_objective output; disturbance_state_out output; disturbance_margins output
function [selected_torques_n_m, cbf_torque_upper_bounds, cbf_active, qp_status, qp_objective, disturbance_state_out, disturbance_margins] = MF_CBF_QP_TorqueAllocator(dt_s, kappa, dot_kappa, kappa_valid, input_gains, previous_applied_torques_n_m, nominal_torques_n_m, base_torques_n_m, wheel_limits_n_m, front_steers_rad, total_torque_n_m, control_mz_n_m)

% CBF-QP 安全扭矩分配模块
%
% 本模块完成：
% 1）滑移率动力学扰动估计；
% 2）CBF滑移安全扭矩上界计算；
% 3）考虑前轮转角的横摆力矩系数计算；
% 4）四轮扭矩QP优化分配。

persistent disturbance_state

if isempty(disturbance_state)
    disturbance_state = zeros(1, 4);
end

%% 输入整理

dt = max(double(dt_s), 0.0);

kappa_vec = row4_local(kappa);
dot_kappa_vec = row4_local(dot_kappa);
valid_vec = row4_local(kappa_valid);
gain_vec = row4_local(input_gains);
applied_vec = row4_local(previous_applied_torques_n_m);
nominal_vec = row4_local(nominal_torques_n_m);
base_vec = row4_local(base_torques_n_m);
limit_vec = row4_local(wheel_limits_n_m);

total_target = double(total_torque_n_m);
yaw_target = double(control_mz_n_m);

steer_input = double(front_steers_rad);

if numel(steer_input) >= 2
    delta_l = steer_input(1);
    delta_r = steer_input(2);
else
    delta_l = steer_input(1);
    delta_r = steer_input(1);
end

%% 轮端限幅整理

wheel_limits = zeros(1, 4);
base_torques = zeros(1, 4);
nominal_torques = zeros(1, 4);

for index = 1:4

    wheel_limits(index) = max(0.0, limit_vec(index));

    base_torques(index) = clamp_local(base_vec(index), 0.0, wheel_limits(index));

    nominal_torques(index) = clamp_local(nominal_vec(index), 0.0, wheel_limits(index));
end

%% 一、等效扰动估计

% 滑移率动力学：
% dot(kappa_i) = g_i * T_i + d_i
%
% 等效扰动估计：
% d_i = dot(kappa_i) - g_i * T_i

disturbance_margins = zeros(1, 4);
alpha_disturbance = first_order_alpha_local(dt, 0.15);

for index = 1:4

    gain = gain_vec(index);

    if valid_vec(index) > 0.5 && isfinite(gain)

        raw_estimate = dot_kappa_vec(index) - gain * applied_vec(index);

        disturbance_state(index) = disturbance_state(index) + ...
            alpha_disturbance * (raw_estimate - disturbance_state(index));

        residual = raw_estimate - disturbance_state(index);

    else

        residual = 0.0;
    end

    % 扰动估计不确定性裕度。
    disturbance_margins(index) = clamp_local(0.05 + 0.05 * abs(residual), 0.05, 5.0);
end

disturbance_state_out = disturbance_state;

%% 二、CBF滑移安全扭矩上界计算

% 安全函数：
% h_i = kappa_max - kappa_i
%
% CBF条件：
% dot(h_i) + gamma*h_i >= 0
%
% 由 dot(kappa_i) = g_i*T_i + d_i 可得：
% g_i*T_i + d_i + margin_i <= gamma*(kappa_max - kappa_i)
%
% 因此：
% T_i <= [gamma*(kappa_max-kappa_i) - d_i - margin_i] / g_i

kappa_max = 0.25;
cbf_gamma = 15.0;

cbf_torque_upper_bounds = zeros(1, 4);
cbf_active = zeros(1, 4);

for index = 1:4

    gain = gain_vec(index);

    if valid_vec(index) > 0.5 && isfinite(gain) && isfinite(kappa_vec(index))

        upper = (cbf_gamma * (kappa_max - kappa_vec(index)) ...
            - disturbance_state(index) ...
            - disturbance_margins(index)) / gain;

        if ~isfinite(upper)
            upper = wheel_limits(index);
        end

        upper = clamp_local(upper, 0.0, wheel_limits(index));

    else

        upper = wheel_limits(index);
    end

    cbf_torque_upper_bounds(index) = upper;

    % 若CBF上界低于基线扭矩，说明安全约束实际参与限幅。
    if upper < base_torques(index) - 1.0e-6
        cbf_active(index) = 1.0;
    end
end

%% 三、考虑前轮转角的横摆力矩映射系数

% 车辆几何参数。
lf = 2.043;
lr = 1.362;

track_front = 2.39;
track_rear = 2.33;

radius_front = 0.834;
radius_rear = 0.94;

% 当前QP只考虑轮端纵向驱动力产生的横摆力矩。
% 对前轮，驱动力方向随转角变化：
% F_x_body = F_i*cos(delta_i)
% F_y_body = F_i*sin(delta_i)
%
% 横摆力矩：
% M_z_i = x_i*F_y_body - y_i*F_x_body
%
% 因为 F_i = T_i/r_i，所以：
% yaw_coeff_i = (x_i*sin(delta_i) - y_i*cos(delta_i)) / r_i

yaw_coefficients = zeros(1, 4);

% 左前轮：x = lf, y = +track_front/2。
yaw_coefficients(1) = (lf * sin(delta_l) - 0.5 * track_front * cos(delta_l)) / radius_front;

% 右前轮：x = lf, y = -track_front/2。
yaw_coefficients(2) = (lf * sin(delta_r) + 0.5 * track_front * cos(delta_r)) / radius_front;

% 左后轮：x = -lr, y = +track_rear/2, delta = 0。
% 因为 sin(0)=0，所以 lr 项不直接进入纵向力横摆力矩。
yaw_coefficients(3) = -0.5 * track_rear / radius_rear;

% 右后轮：x = -lr, y = -track_rear/2, delta = 0。
yaw_coefficients(4) = 0.5 * track_rear / radius_rear;

%% 四、QP四轮扭矩优化分配

lower_bounds = zeros(1, 4);

[qp_torques, qp_status, qp_objective] = solve_torque_qp_local( ...
    nominal_torques, ...
    total_target, ...
    yaw_target, ...
    lower_bounds, ...
    cbf_torque_upper_bounds, ...
    yaw_coefficients);

%% 五、QP失败时安全降级

if qp_status > 0.5

    selected_torques_n_m = qp_torques;

else

    selected_torques_n_m = zeros(1, 4);

    for index = 1:4
        selected_torques_n_m(index) = clamp_local(base_torques(index), 0.0, cbf_torque_upper_bounds(index));
    end
end

end


function [solution, status, objective] = solve_torque_qp_local(nominal, total_target, yaw_target, lower, upper, yaw)

% 四轮扭矩边界约束QP求解器
%
% 决策变量：
% T = [T1, T2, T3, T4]
%
% 目标函数：
% J = 0.5*w_nominal*sum((T_i - T_nom_i)^2)
%   + 0.5*w_total*(sum(T_i) - T_total_ref)^2
%   + 0.5*w_yaw*(yaw*T' - Mz_ref)^2
%   + regularization*sum(T_i^2)
%
% 约束：
% lower_i <= T_i <= upper_i
%
% 由于只有4个决策变量，这里采用主动集枚举方法，
% 每个变量枚举为下界、自由、上界三种状态。

status = -1.0;
objective = NaN;
solution = zeros(1, 4);

%% 可行性预检查

for index = 1:4
    if upper(index) < lower(index) || ~isfinite(upper(index)) || ~isfinite(lower(index))
        return;
    end
end

%% 权重参数

weight_nominal = 1.0;
weight_total = 1.12;
weight_yaw = 0.02;
regularization = 1.0e-6;

%% 构造二次型矩阵和线性项

H = zeros(4, 4);
linear = zeros(1, 4);

for row = 1:4

    for col = 1:4

        % 总扭矩项对 Hessian 的贡献。
        % 横摆力矩项对 Hessian 的贡献。
        H(row, col) = H(row, col) + weight_total + weight_yaw * yaw(row) * yaw(col);
    end

    % 名义扭矩跟踪项和正则化项。
    H(row, row) = H(row, row) + weight_nominal + 2.0 * regularization;

    % 线性项。
    linear(row) = linear(row) ...
        - weight_nominal * nominal(row) ...
        - weight_total * total_target ...
        - weight_yaw * yaw_target * yaw(row);
end

%% 主动集枚举

best_objective = Inf;

% -1：固定在下界；
%  0：自由变量；
%  1：固定在上界。
states = [-1.0, 0.0, 1.0];

for i1 = 1:3
    for i2 = 1:3
        for i3 = 1:3
            for i4 = 1:3

                activity = [states(i1), states(i2), states(i3), states(i4)];

                candidate = zeros(1, 4);
                free_indices = zeros(1, 4);
                nfree = 0;

                %% 设置固定变量并记录自由变量

                for index = 1:4

                    if activity(index) < -0.5

                        candidate(index) = lower(index);

                    elseif activity(index) > 0.5

                        candidate(index) = upper(index);

                    else

                        nfree = nfree + 1;
                        free_indices(nfree) = index;
                    end
                end

                %% 求解自由变量

                if nfree > 0

                    A = zeros(4, 4);
                    b = zeros(1, 4);

                    for rr = 1:nfree

                        row = free_indices(rr);
                        fixed_contribution = 0.0;

                        for col = 1:4
                            if activity(col) ~= 0.0
                                fixed_contribution = fixed_contribution + H(row, col) * candidate(col);
                            end
                        end

                        b(rr) = -linear(row) - fixed_contribution;

                        for cc = 1:nfree
                            A(rr, cc) = H(row, free_indices(cc));
                        end
                    end

                    [free_solution, ok] = solve_linear_system4_local(A, b, nfree);

                    if ok <= 0.5
                        continue;
                    end

                    for rr = 1:nfree
                        candidate(free_indices(rr)) = free_solution(rr);
                    end
                end

                %% 可行性检查

                feasible = 1.0;

                for index = 1:4

                    if candidate(index) < lower(index) - 1.0e-7 || ...
                            candidate(index) > upper(index) + 1.0e-7 || ...
                            ~isfinite(candidate(index))

                        feasible = 0.0;
                    end

                    candidate(index) = clamp_local(candidate(index), lower(index), upper(index));
                end

                if feasible <= 0.5
                    continue;
                end

                %% 计算目标函数

                obj = quadratic_objective_local(candidate, H, linear);

                if obj < best_objective

                    best_objective = obj;
                    solution = candidate;
                    status = 1.0;
                    objective = obj;
                end
            end
        end
    end
end

end


function [x, ok] = solve_linear_system4_local(A, b, n)

% 求解最多4维线性方程组 A*x=b。
% 采用带部分主元选择的高斯消元法。

x = zeros(1, 4);
ok = 1.0;

if n == 0
    return;
end

aug = zeros(4, 5);

for row = 1:n

    for col = 1:n
        aug(row, col) = A(row, col);
    end

    aug(row, n + 1) = b(row);
end

%% 前向消元

for col = 1:n

    pivot_row = col;
    pivot_abs = abs(aug(col, col));

    for row = col:n
        if abs(aug(row, col)) > pivot_abs
            pivot_abs = abs(aug(row, col));
            pivot_row = row;
        end
    end

    if pivot_abs <= 1.0e-12 || ~isfinite(pivot_abs)
        ok = 0.0;
        return;
    end

    if pivot_row ~= col

        temp = aug(col, :);
        aug(col, :) = aug(pivot_row, :);
        aug(pivot_row, :) = temp;
    end

    for row = col + 1:n

        factor = aug(row, col) / aug(col, col);

        if factor ~= 0.0

            for entry = col:n + 1
                aug(row, entry) = aug(row, entry) - factor * aug(col, entry);
            end
        end
    end
end

%% 回代

for row = n:-1:1

    residual = aug(row, n + 1);

    for col = row + 1:n
        residual = residual - aug(row, col) * x(col);
    end

    pivot = aug(row, row);

    if abs(pivot) <= 1.0e-12
        ok = 0.0;
        return;
    end

    x(row) = residual / pivot;

    if ~isfinite(x(row))
        ok = 0.0;
        return;
    end
end

end


function value = quadratic_objective_local(torques, H, linear)

% QP目标函数：
% J = 0.5*T*H*T' + linear*T'

value = 0.0;

for row = 1:4

    for col = 1:4
        value = value + 0.5 * torques(row) * H(row, col) * torques(col);
    end

    value = value + linear(row) * torques(row);
end

end


function output = row4_local(values)

% 将输入信号整理为 1×4 行向量。

input_values = double(values);
output = zeros(1, 4);

for index = 1:4
    output(index) = input_values(index);
end

end


function alpha = first_order_alpha_local(dt, time_constant_s)

% 一阶低通滤波系数。

if dt <= 0.0 || time_constant_s <= 0.0
    alpha = 1.0;
else
    alpha = dt / (time_constant_s + dt);
end

end


function value = clamp_local(value_in, lower, upper)

% 数值限幅函数。

value = min(max(double(value_in), double(lower)), double(upper));

end

== matlab function tractor_mu/软土扭矩分配/牵引效率评价计算 ==
  data: dt_s input; eta_wg_E output; drawbar_power_w input; wheel_power_w input; E_wg output; E_w output; drawbar_force input
function [eta_wg_E, E_wg, E_w] = MF_EnergyWeightedTractionEfficiency(dt_s, drawbar_power_w, wheel_power_w, drawbar_force)

persistent E_wg_state E_w_state

if isempty(E_wg_state)
    E_wg_state = 0.0;
    E_w_state = 0.0;
end

dt = max(double(dt_s), 0.0);

epsilon_E = 1.0;   % 防止低能量窗口除零，可根据功率量级调整

%window_enable = wheel_power_w > 100 && drawbar_force > 10;
window_enable = 1;

if double(window_enable) > 0.5
    E_wg_state = E_wg_state + max(0.0, double(drawbar_power_w)) * dt;
    E_w_state = E_w_state + max(0.0, double(wheel_power_w)) * dt;
end

eta_wg_E = E_wg_state / (E_w_state + epsilon_E);

E_wg = E_wg_state;
E_w = E_w_state;

end
